simulink model "MMC_1ph_Grid_ArmLeaders_EnergyBalancing_v3_1A"  (R2024a)
settings: Solver=FixedStepDiscrete  StartTime=0.0  StopTime=1  FixedStep=Ts  RelTol=1e-3
PreLoadFcn:
  | VDC=800; N=8; C=2.2e-3; vo=100; W_nom=0.5*C*N*vo^2;
  | Larm=5e-3; Rarm=0.5; f=50;
  | Vg_rms=230; Vg_pk=Vg_rms*sqrt(2); Lg=2e-3; Rg=0.1;
  | Pstar=1500; Qstar=0;
  | fsw=1250; Ts=1e-5; Ts_ctrl=1e-4; Cf=10e-6; Rf=10;
InitFcn:
  | VDC=800; N=8; C=2.2e-3; vo=100; W_nom=0.5*C*N*vo^2;
  | Larm=5e-3; Rarm=0.5; f=50;
  | Vg_rms=230; Vg_pk=Vg_rms*sqrt(2); Lg=2e-3; Rg=0.1;
  | Pstar=1500; Qstar=0;
  | fsw=1250; Ts=1e-5; Ts_ctrl=1e-4; Cf=10e-6; Rf=10;
libraries: spsHalfBridgeMMCLib x16, spsSeriesRLCBranchLib x4, spsCurrentMeasurementLib x3, spsGroundLib x2, spsDCVoltageSourceLib x2, spsACVoltageSourceLib x1, spspowerguiLib x1, spsVoltageMeasurementLib x1
(part 1 of 2)
settings Model: Creator=Dell  LastModifiedBy=Dell
settings SolverCC: AutoInsertRateTranBlk=on

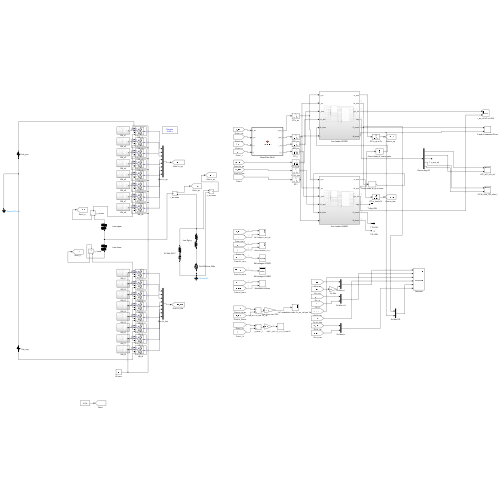
[thumbnail: Simulink's stored preview of the top-level diagram]
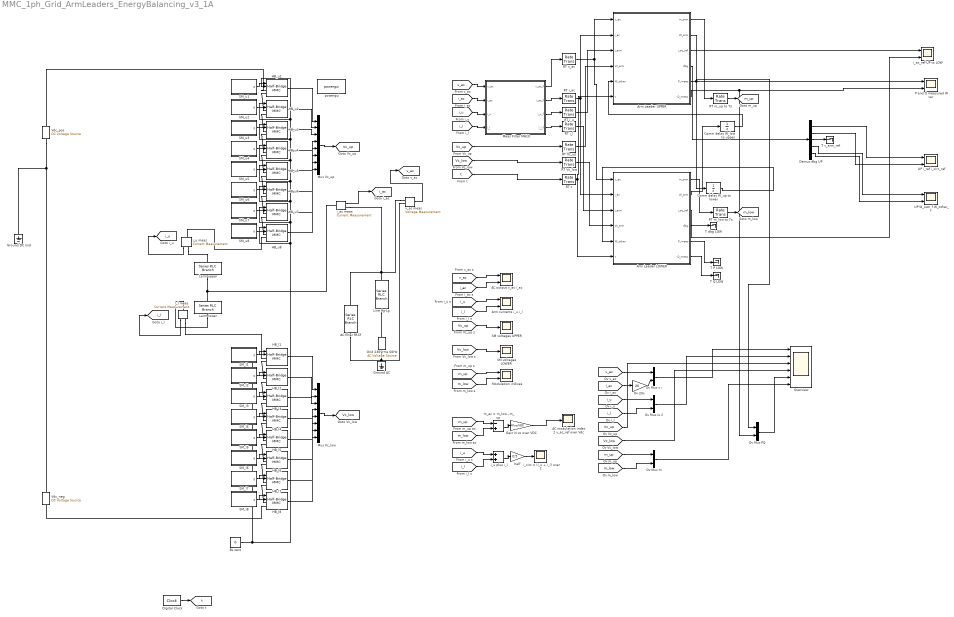
== system MMC_1ph_Grid_ArmLeaders_EnergyBalancing_v3_1A ==
  AC filter Rf-Cf : spsSeriesRLCBranchLib/Series RLC Branch  LConnTagsString=__new0  RConnTagsString=__new0  BranchType=RC  Resistance=Rf  Inductance=1e-3  SetiL0=off  InitialCurrent=0  Capacitance=Cf  Setx0=off  InitialVoltage=0  Measurements=None
  AC modulation index 2 v_ac_ref over Vdc : Scope
  AC output v_ac i_ac : Scope  NumInputPorts=2
  Arm Leader LOWER : Subsystem
  Arm Leader UPPER : Subsystem
  Arm currents i_u i_l : Scope  NumInputPorts=2
  BL zero : Constant  Value=0
  Comm delay W_low to upper : UnitDelay  InitialCondition=W_nom  SampleTime=Ts_ctrl  HasFrameUpgradeWarning=on
  Comm delay W_up to lower : UnitDelay  InitialCondition=W_nom  SampleTime=Ts_ctrl  HasFrameUpgradeWarning=on
  Demux dbg UP : Demux  Outputs=5
  Digital Clock : DigitalClock  SampleTime=Ts
  Gain N vo over VDC : Gain  Gain=N*vo/VDC
  Grid 230Vrms 50Hz : spsACVoltageSourceLib/AC Voltage Source  Amplitude=Vg_pk  Phase=0  Frequency=f  SampleTime=0  Measurements=None  BusType=swing  Pref=10e3  Qref=0  Qmin=-inf  Qmax=+inf
  Ground AC : spsGroundLib/Ground  LConnTagsString=a
  Ground DC mid : spsGroundLib/Ground  LConnTagsString=a
  HB_l{1..8} (8 alike) : spsHalfBridgeMMCLib/Half-Bridge MMC  ModelType=Switching devices  n=1  C=C  Vc_Initial=vo  Ron=1e-3  Rs=1e6  Cs=inf  Ron_Diode=1e-3  Rs_Diode=1e6  Cs_Diode=inf  Vf_Diode=1e-3  Rs_CurrentSource=inf  Ts=Ts
  HB_u{1..8} (8 alike) : spsHalfBridgeMMCLib/Half-Bridge MMC  ModelType=Switching devices  n=1  C=C  Vc_Initial=vo  Ron=1e-3  Rs=1e6  Cs=inf  Ron_Diode=1e-3  Rs_Diode=1e6  Cs_Diode=inf  Vf_Diode=1e-3  Rs_CurrentSource=inf  Ts=Ts
  Larm lower : spsSeriesRLCBranchLib/Series RLC Branch  LConnTagsString=__new0  RConnTagsString=__new0  BranchType=RL  Resistance=Rarm  Inductance=Larm  SetiL0=off  InitialCurrent=0  Capacitance=1e-6  Setx0=off  InitialVoltage=0  Measurements=None
  Larm upper : spsSeriesRLCBranchLib/Series RLC Branch  LConnTagsString=__new0  RConnTagsString=__new0  BranchType=RL  Resistance=Rarm  Inductance=Larm  SetiL0=off  InitialCurrent=0  Capacitance=1e-6  Setx0=off  InitialVoltage=0  Measurements=None
  Line Rg-Lg : spsSeriesRLCBranchLib/Series RLC Branch  LConnTagsString=__new0  RConnTagsString=__new0  BranchType=RL  Resistance=Rg  Inductance=Lg  SetiL0=off  InitialCurrent=0  Capacitance=1e-6  Setx0=off  InitialVoltage=0  Measurements=None
  Meas Filter MA10 : MATLAB Function  TreatAsAtomicUnit=on
  Modulation indices : Scope  NumInputPorts=2
  Mux Vc_low : Mux  Inputs=8
  Mux Vc_up : Mux  Inputs=8
  Ov 20x : Gain  Gain=20
  Ov Mux PQ : Mux  Inputs=2
  Ov Mux iu il : Mux  Inputs=2
  Ov Mux m : Mux  Inputs=2
  Ov Mux v i : Mux  Inputs=2
  Overview : Scope  NumInputPorts=6
  P and Q measured W var : Scope  NumInputPorts=2
  RT Vc_low : RateTransition  OutPortSampleTime=Ts_ctrl
  RT Vc_up : RateTransition  OutPortSampleTime=Ts_ctrl
  RT i_ac : RateTransition  OutPortSampleTime=Ts_ctrl
  RT i_l : RateTransition  OutPortSampleTime=Ts_ctrl
  RT i_u : RateTransition  OutPortSampleTime=Ts_ctrl
  RT m_low to Ts : RateTransition  Deterministic=off  OutPortSampleTime=Ts
  RT m_up to Ts : RateTransition  Deterministic=off  OutPortSampleTime=Ts
  RT t : RateTransition  OutPortSampleTime=Ts_ctrl
  RT v_ac : RateTransition  OutPortSampleTime=Ts_ctrl
  SM voltages LOWER : Scope
  SM voltages UPPER : Scope
  SM_l1 : Subsystem
  SM_l2 : Subsystem
  SM_l3 : Subsystem
  SM_l4 : Subsystem
  SM_l5 : Subsystem
  SM_l6 : Subsystem
  SM_l7 : Subsystem
  SM_l8 : Subsystem
  SM_u1 : Subsystem
  SM_u2 : Subsystem
  SM_u3 : Subsystem
  SM_u4 : Subsystem
  SM_u5 : Subsystem
  SM_u6 : Subsystem
  SM_u7 : Subsystem
  SM_u8 : Subsystem
  T P LOW : Terminator
  T Q LOW : Terminator
  T dbg LOW : Terminator
  T v_arm_ref : Terminator
  UP W_own_f W_other_f : Scope  NumInputPorts=2
  UP i_ref i_circ_ref : Scope  NumInputPorts=2
  Vdc_neg : spsDCVoltageSourceLib/DC Voltage Source  Amplitude=VDC/2  Measurements=None
  Vdc_pos : spsDCVoltageSourceLib/DC Voltage Source  Amplitude=VDC/2  Measurements=None
  half : Gain  Gain=0.5
  i_ac meas : spsCurrentMeasurementLib/Current Measurement  PhasorSimulation=off  OutputType=Complex  PSBequivalent=0
  i_ac_ref UP vs LOW : Scope  NumInputPorts=2
  i_circ = (i_u + i_l) over 2 : Scope
  i_l meas : spsCurrentMeasurementLib/Current Measurement  PhasorSimulation=off  OutputType=Complex  PSBequivalent=0
  i_u meas : spsCurrentMeasurementLib/Current Measurement  PhasorSimulation=off  OutputType=Complex  PSBequivalent=0
  i_u plus i_l : Sum
  m_ac = m_low - m_up : Sum  Inputs=-+
  powergui : spspowerguiLib/powergui  Priority=1  SimulationMode=Discrete  SampleTime=Ts  frequency=50  Iterations=50  frequencyindice=50  Pbase=100e6  ErrMax=1e-4  UnitsV=kV  UnitsW=MW  buscounter=0  FunctionMessages=off  echomessages=off  EnableUseOfTLC=off  CurrentSourceSwitches=off  DisableSnubberDevices=off  DisableRonSwitches=off  DisableVfSwitches=off  DisplayEquations=off  AutomaticDiscreteSolvers=off  SolverType=Tustin/Backward Euler (TBE)  Interpol=off  ExternalGateDelay=off  methode=off  Ts=100  x0status=blocks  SPID=on  SwTol=0  HookPort=off  NonlinearTolerance=1e-4  nMaxIteration=100  ContinueOnMaxIteration=off  RestoreLinks=warning  ResistiveCurrentMeasurement=off  Frange=[0:2:500]  Ylog=off  Xlog=on  ShowGrid=off  save=off  variable=ZData  structure=0  ZoomFFT=off  StartTime=0.0  cycles=1  DisplayStyle=1  fundamental=50  FreqAxis=off  MaxFrequency=1000  frequencyindicesteady=1  RmsSteady=1  display=off
  v_ac meas : spsVoltageMeasurementLib/Voltage Measurement  PhasorSimulation=off  OutputType=Complex  PSBequivalent=0
  tag scope: Vc_low=global, Vc_up=global, i_ac=global, i_l=global, i_u=global, m_low=global, m_up=global, t=global, v_ac=global
  wires:
  v_ac meas/1 -> [v_ac]
  i_ac meas/1 -> [i_ac]
  i_u meas/1 -> [i_u]
  i_l meas/1 -> [i_l]
  BL zero/1 -> HB_u1/2, HB_u2/2, HB_u3/2, HB_u4/2, HB_u5/2, HB_u6/2, HB_u7/2, HB_u8/2, HB_l1/2, HB_l2/2, HB_l3/2, HB_l4/2, HB_l5/2, HB_l6/2, HB_l7/2, HB_l8/2
  HB_u1/1 -> Mux Vc_up/1
  HB_l1/1 -> Mux Vc_low/1
  HB_u2/1 -> Mux Vc_up/2
  HB_l2/1 -> Mux Vc_low/2
  HB_u3/1 -> Mux Vc_up/3
  HB_l3/1 -> Mux Vc_low/3
  HB_u4/1 -> Mux Vc_up/4
  HB_l4/1 -> Mux Vc_low/4
  HB_u5/1 -> Mux Vc_up/5
  HB_l5/1 -> Mux Vc_low/5
  HB_u6/1 -> Mux Vc_up/6
  HB_l6/1 -> Mux Vc_low/6
  HB_u7/1 -> Mux Vc_up/7
  HB_l7/1 -> Mux Vc_low/7
  HB_u8/1 -> Mux Vc_up/8
  HB_l8/1 -> Mux Vc_low/8
  Mux Vc_up/1 -> [Vc_up]
  Mux Vc_low/1 -> [Vc_low]
  Digital Clock/1 -> [t]
  SM_u1/1(g) -> HB_u1/1
  SM_l1/1(g) -> HB_l1/1
  SM_u2/1(g) -> HB_u2/1
  SM_l2/1(g) -> HB_l2/1
  SM_u3/1(g) -> HB_u3/1
  SM_l3/1(g) -> HB_l3/1
  SM_u4/1(g) -> HB_u4/1
  SM_l4/1(g) -> HB_l4/1
  SM_u5/1(g) -> HB_u5/1
  SM_l5/1(g) -> HB_l5/1
  SM_u6/1(g) -> HB_u6/1
  SM_l6/1(g) -> HB_l6/1
  SM_u7/1(g) -> HB_u7/1
  SM_l7/1(g) -> HB_l7/1
  SM_u8/1(g) -> HB_u8/1
  SM_l8/1(g) -> HB_l8/1
  [v_ac] -> Meas Filter MA10/1(v_ac)
  [i_ac] -> Meas Filter MA10/2(i_ac)
  [i_u] -> Meas Filter MA10/3(i_u)
  [i_l] -> Meas Filter MA10/4(i_l)
  Meas Filter MA10/1(v_ac_f) -> RT v_ac/1
  Meas Filter MA10/2(i_ac_f) -> RT i_ac/1
  Meas Filter MA10/3(i_u_f) -> RT i_u/1
  Meas Filter MA10/4(i_l_f) -> RT i_l/1
  [Vc_up] -> RT Vc_up/1
  [Vc_low] -> RT Vc_low/1
  [t] -> RT t/1
  RT v_ac/1 -> Arm Leader LOWER/1(v_ac), Arm Leader UPPER/1(v_ac)
  RT i_ac/1 -> Arm Leader UPPER/2(i_ac), Arm Leader LOWER/2(i_ac)
  RT i_u/1 -> Arm Leader UPPER/3(i_arm)
  RT i_l/1 -> Arm Leader LOWER/3(i_arm)
  RT Vc_up/1 -> Arm Leader UPPER/4(Vc_arm)
  RT Vc_low/1 -> Arm Leader LOWER/4(Vc_arm)
  RT t/1 -> Arm Leader UPPER/6(t), Arm Leader LOWER/6(t)
  Arm Leader UPPER/2(W_arm) -> Comm delay W_up to lower/1
  Comm delay W_up to lower/1 -> Arm Leader LOWER/5(W_other)
  Arm Leader LOWER/2(W_arm) -> Comm delay W_low to upper/1
  Comm delay W_low to upper/1 -> Arm Leader UPPER/5(W_other)
  Arm Leader UPPER/1(m_arm) -> RT m_up to Ts/1
  RT m_up to Ts/1 -> [m_up]
  Arm Leader LOWER/1(m_arm) -> RT m_low to Ts/1
  RT m_low to Ts/1 -> [m_low]
  [v_ac] -> AC output v_ac i_ac/1
  [i_ac] -> AC output v_ac i_ac/2
  [i_u] -> Arm currents i_u i_l/1
  [i_l] -> Arm currents i_u i_l/2
  [Vc_up] -> SM voltages UPPER/1
  [Vc_low] -> SM voltages LOWER/1
  [m_up] -> Modulation indices/1
  [m_low] -> Modulation indices/2
  [m_up] -> m_ac = m_low - m_up/1
  [m_low] -> m_ac = m_low - m_up/2
  m_ac = m_low - m_up/1 -> Gain N vo over VDC/1
  Gain N vo over VDC/1 -> AC modulation index 2 v_ac_ref over Vdc/1
  [i_u] -> i_u plus i_l/1
  [i_l] -> i_u plus i_l/2
  i_u plus i_l/1 -> half/1
  half/1 -> i_circ = (i_u + i_l) over 2/1
  Arm Leader UPPER/5(P_meas) -> P and Q measured W var/1, Ov Mux PQ/1
  Arm Leader UPPER/6(Q_meas) -> P and Q measured W var/2, Ov Mux PQ/2
  Arm Leader UPPER/3(i_ac_ref) -> i_ac_ref UP vs LOW/1
  Arm Leader LOWER/3(i_ac_ref) -> i_ac_ref UP vs LOW/2
  Arm Leader UPPER/4(dbg) -> Demux dbg UP/1
  Demux dbg UP/1 -> UP i_ref i_circ_ref/1
  Demux dbg UP/2 -> UP i_ref i_circ_ref/2
  Demux dbg UP/3 -> T v_arm_ref/1
  Demux dbg UP/4 -> UP W_own_f W_other_f/1
  Demux dbg UP/5 -> UP W_own_f W_other_f/2
  Arm Leader LOWER/4(dbg) -> T dbg LOW/1
  Arm Leader LOWER/5(P_meas) -> T P LOW/1
  Arm Leader LOWER/6(Q_meas) -> T Q LOW/1
  [v_ac] -> Ov Mux v i/1
  [i_ac] -> Ov 20x/1
  Ov 20x/1 -> Ov Mux v i/2
  [i_u] -> Ov Mux iu il/1
  [i_l] -> Ov Mux iu il/2
  [m_up] -> Ov Mux m/1
  [m_low] -> Ov Mux m/2
  Ov Mux v i/1 -> Overview/1
  Ov Mux iu il/1 -> Overview/2
  [Vc_up] -> Overview/3
  [Vc_low] -> Overview/4
  Ov Mux PQ/1 -> Overview/5
  Ov Mux m/1 -> Overview/6
  connections:
  HB_u1/LConn1 -- Vdc_pos/RConn1
  Vdc_pos/LConn1 -- Ground DC mid/LConn1 -- Vdc_neg/RConn1
  HB_u1/LConn2 -- HB_u2/LConn1
  HB_l1/LConn2 -- HB_l2/LConn1
  HB_u2/LConn2 -- HB_u3/LConn1
  HB_l2/LConn2 -- HB_l3/LConn1
  HB_u3/LConn2 -- HB_u4/LConn1
  HB_l3/LConn2 -- HB_l4/LConn1
  HB_u4/LConn2 -- HB_u5/LConn1
  HB_l4/LConn2 -- HB_l5/LConn1
  HB_u5/LConn2 -- HB_u6/LConn1
  HB_l5/LConn2 -- HB_l6/LConn1
  HB_u6/LConn2 -- HB_u7/LConn1
  HB_l6/LConn2 -- HB_l7/LConn1
  HB_u7/LConn2 -- HB_u8/LConn1
  HB_l7/LConn2 -- HB_l8/LConn1
  HB_u8/LConn2 -- i_u meas/LConn1
  i_u meas/RConn1 -- Larm upper/LConn1
  Larm upper/RConn1 -- i_ac meas/LConn1 -- Larm lower/LConn1
  Larm lower/RConn1 -- i_l meas/LConn1
  i_l meas/RConn1 -- HB_l1/LConn1
  HB_l8/LConn2 -- Vdc_neg/LConn1
  v_ac meas/LConn1 -- i_ac meas/RConn1 -- Line Rg-Lg/LConn1 -- AC filter Rf-Cf/LConn1
  Line Rg-Lg/RConn1 -- Grid 230Vrms 50Hz/RConn1
  Grid 230Vrms 50Hz/LConn1 -- AC filter Rf-Cf/RConn1 -- v_ac meas/LConn2 -- Ground AC/LConn1

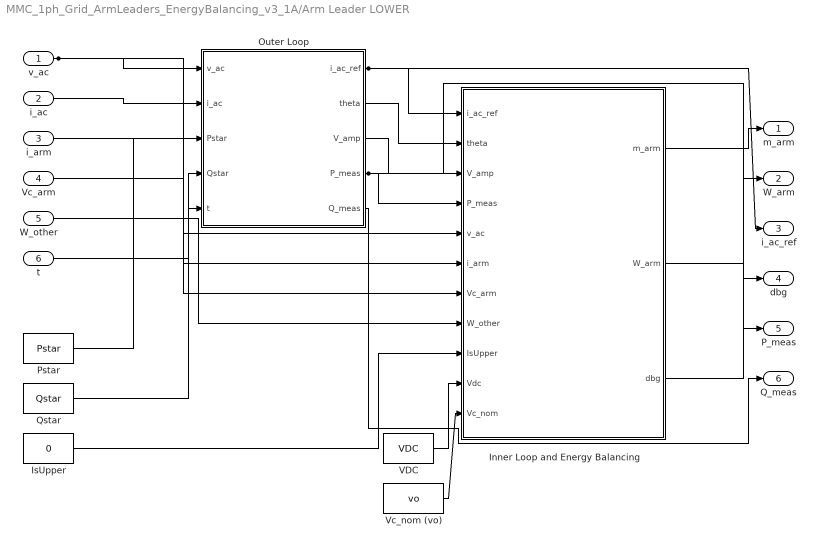
== system MMC_1ph_Grid_ArmLeaders_EnergyBalancing_v3_1A/Arm Leader LOWER ==
  v_ac : Inport
  i_ac : Inport  Port=2
  i_arm : Inport  Port=3
  Vc_arm : Inport  Port=4
  W_other : Inport  Port=5
  t : Inport  Port=6
  Inner Loop and Energy Balancing : MATLAB Function  TreatAsAtomicUnit=on
  IsUpper : Constant  Value=0
  Outer Loop : MATLAB Function  TreatAsAtomicUnit=on
  Pstar : Constant  Value=Pstar
  Qstar : Constant  Value=Qstar
  VDC : Constant  Value=VDC
  Vc_nom (vo) : Constant  Value=vo
  m_arm : Outport
  W_arm : Outport  Port=2
  i_ac_ref : Outport  Port=3
  dbg : Outport  Port=4
  P_meas : Outport  Port=5
  Q_meas : Outport  Port=6
  wires:
  v_ac/1 -> Outer Loop/1(v_ac), Inner Loop and Energy Balancing/5(v_ac)
  i_ac/1 -> Outer Loop/2(i_ac)
  Pstar/1 -> Outer Loop/3(Pstar)
  Qstar/1 -> Outer Loop/4(Qstar)
  t/1 -> Outer Loop/5(t)
  Outer Loop/1(i_ac_ref) -> Inner Loop and Energy Balancing/1(i_ac_ref), i_ac_ref/1
  Outer Loop/2(theta) -> Inner Loop and Energy Balancing/2(theta)
  Outer Loop/3(V_amp) -> Inner Loop and Energy Balancing/3(V_amp)
  Outer Loop/4(P_meas) -> Inner Loop and Energy Balancing/4(P_meas), P_meas/1
  Outer Loop/5(Q_meas) -> Q_meas/1
  i_arm/1 -> Inner Loop and Energy Balancing/6(i_arm)
  Vc_arm/1 -> Inner Loop and Energy Balancing/7(Vc_arm)
  W_other/1 -> Inner Loop and Energy Balancing/8(W_other)
  IsUpper/1 -> Inner Loop and Energy Balancing/9(IsUpper)
  VDC/1 -> Inner Loop and Energy Balancing/10(Vdc)
  Vc_nom (vo)/1 -> Inner Loop and Energy Balancing/11(Vc_nom)
  Inner Loop and Energy Balancing/1(m_arm) -> m_arm/1
  Inner Loop and Energy Balancing/2(W_arm) -> W_arm/1
  Inner Loop and Energy Balancing/3(dbg) -> dbg/1

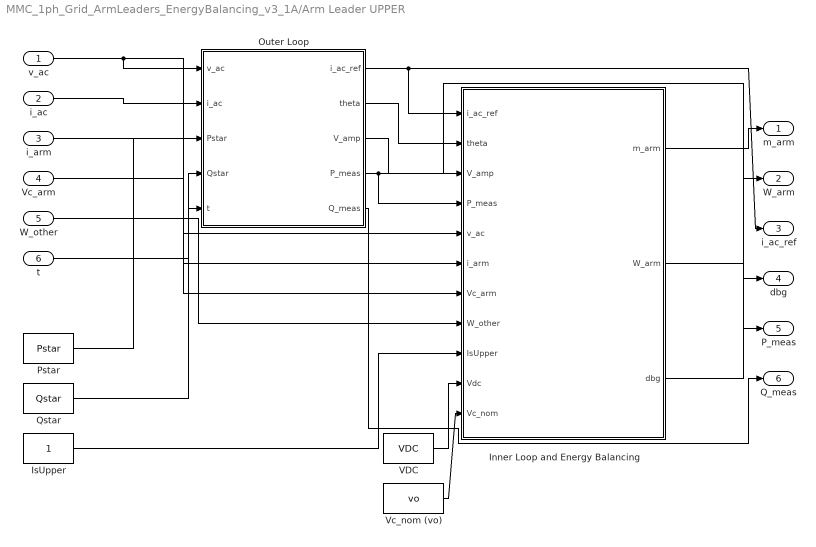
== system MMC_1ph_Grid_ArmLeaders_EnergyBalancing_v3_1A/Arm Leader UPPER ==
  v_ac : Inport
  i_ac : Inport  Port=2
  i_arm : Inport  Port=3
  Vc_arm : Inport  Port=4
  W_other : Inport  Port=5
  t : Inport  Port=6
  Inner Loop and Energy Balancing : MATLAB Function  TreatAsAtomicUnit=on
  IsUpper : Constant
  Outer Loop : MATLAB Function  TreatAsAtomicUnit=on
  Pstar : Constant  Value=Pstar
  Qstar : Constant  Value=Qstar
  VDC : Constant  Value=VDC
  Vc_nom (vo) : Constant  Value=vo
  m_arm : Outport
  W_arm : Outport  Port=2
  i_ac_ref : Outport  Port=3
  dbg : Outport  Port=4
  P_meas : Outport  Port=5
  Q_meas : Outport  Port=6
  wires:
  v_ac/1 -> Outer Loop/1(v_ac), Inner Loop and Energy Balancing/5(v_ac)
  i_ac/1 -> Outer Loop/2(i_ac)
  Pstar/1 -> Outer Loop/3(Pstar)
  Qstar/1 -> Outer Loop/4(Qstar)
  t/1 -> Outer Loop/5(t)
  Outer Loop/1(i_ac_ref) -> Inner Loop and Energy Balancing/1(i_ac_ref), i_ac_ref/1
  Outer Loop/2(theta) -> Inner Loop and Energy Balancing/2(theta)
  Outer Loop/3(V_amp) -> Inner Loop and Energy Balancing/3(V_amp)
  Outer Loop/4(P_meas) -> Inner Loop and Energy Balancing/4(P_meas), P_meas/1
  Outer Loop/5(Q_meas) -> Q_meas/1
  i_arm/1 -> Inner Loop and Energy Balancing/6(i_arm)
  Vc_arm/1 -> Inner Loop and Energy Balancing/7(Vc_arm)
  W_other/1 -> Inner Loop and Energy Balancing/8(W_other)
  IsUpper/1 -> Inner Loop and Energy Balancing/9(IsUpper)
  VDC/1 -> Inner Loop and Energy Balancing/10(Vdc)
  Vc_nom (vo)/1 -> Inner Loop and Energy Balancing/11(Vc_nom)
  Inner Loop and Energy Balancing/1(m_arm) -> m_arm/1
  Inner Loop and Energy Balancing/2(W_arm) -> W_arm/1
  Inner Loop and Energy Balancing/3(dbg) -> dbg/1

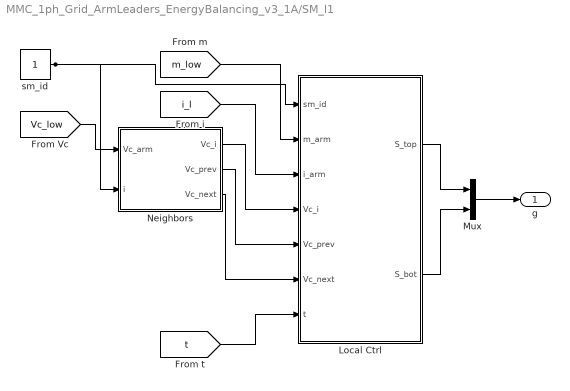
== system MMC_1ph_Grid_ArmLeaders_EnergyBalancing_v3_1A/SM_l1 ==
  Local Ctrl : MATLAB Function  TreatAsAtomicUnit=on
  Mux : Mux  Inputs=2
  Neighbors : MATLAB Function  TreatAsAtomicUnit=on
  sm_id : Constant
  g : Outport
  wires:
  [Vc_low] -> Neighbors/1(Vc_arm)
  sm_id/1 -> Neighbors/2(i), Local Ctrl/1(sm_id)
  [m_low] -> Local Ctrl/2(m_arm)
  [i_l] -> Local Ctrl/3(i_arm)
  Neighbors/1(Vc_i) -> Local Ctrl/4(Vc_i)
  Neighbors/2(Vc_prev) -> Local Ctrl/5(Vc_prev)
  Neighbors/3(Vc_next) -> Local Ctrl/6(Vc_next)
  [t] -> Local Ctrl/7(t)
  Local Ctrl/1(S_top) -> Mux/1
  Local Ctrl/2(S_bot) -> Mux/2
  Mux/1 -> g/1

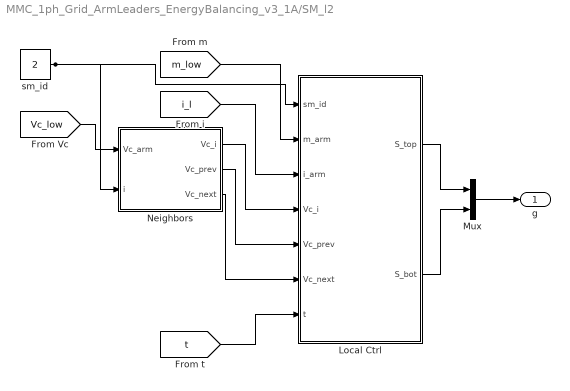
== system MMC_1ph_Grid_ArmLeaders_EnergyBalancing_v3_1A/SM_l2 ==
  Local Ctrl : MATLAB Function  TreatAsAtomicUnit=on
  Mux : Mux  Inputs=2
  Neighbors : MATLAB Function  TreatAsAtomicUnit=on
  sm_id : Constant  Value=2
  g : Outport
  wires:
  [Vc_low] -> Neighbors/1(Vc_arm)
  sm_id/1 -> Neighbors/2(i), Local Ctrl/1(sm_id)
  [m_low] -> Local Ctrl/2(m_arm)
  [i_l] -> Local Ctrl/3(i_arm)
  Neighbors/1(Vc_i) -> Local Ctrl/4(Vc_i)
  Neighbors/2(Vc_prev) -> Local Ctrl/5(Vc_prev)
  Neighbors/3(Vc_next) -> Local Ctrl/6(Vc_next)
  [t] -> Local Ctrl/7(t)
  Local Ctrl/1(S_top) -> Mux/1
  Local Ctrl/2(S_bot) -> Mux/2
  Mux/1 -> g/1

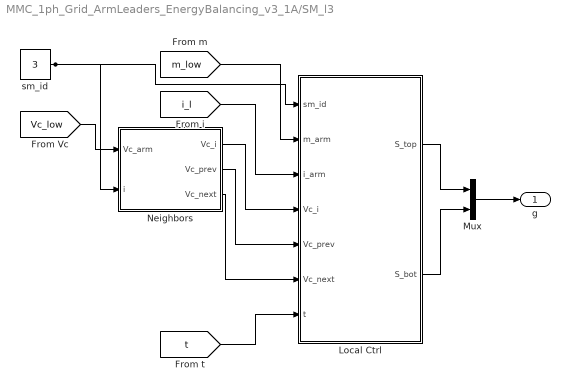
== system MMC_1ph_Grid_ArmLeaders_EnergyBalancing_v3_1A/SM_l3 ==
  Local Ctrl : MATLAB Function  TreatAsAtomicUnit=on
  Mux : Mux  Inputs=2
  Neighbors : MATLAB Function  TreatAsAtomicUnit=on
  sm_id : Constant  Value=3
  g : Outport
  wires:
  [Vc_low] -> Neighbors/1(Vc_arm)
  sm_id/1 -> Neighbors/2(i), Local Ctrl/1(sm_id)
  [m_low] -> Local Ctrl/2(m_arm)
  [i_l] -> Local Ctrl/3(i_arm)
  Neighbors/1(Vc_i) -> Local Ctrl/4(Vc_i)
  Neighbors/2(Vc_prev) -> Local Ctrl/5(Vc_prev)
  Neighbors/3(Vc_next) -> Local Ctrl/6(Vc_next)
  [t] -> Local Ctrl/7(t)
  Local Ctrl/1(S_top) -> Mux/1
  Local Ctrl/2(S_bot) -> Mux/2
  Mux/1 -> g/1

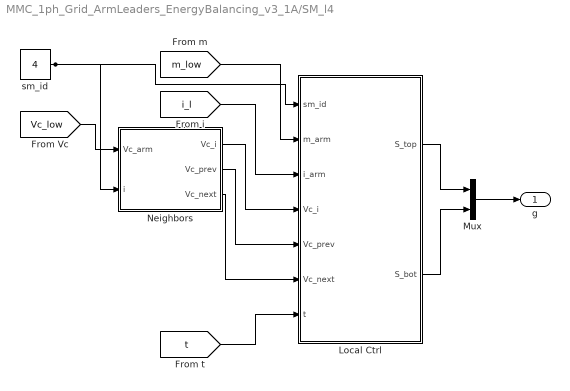
== system MMC_1ph_Grid_ArmLeaders_EnergyBalancing_v3_1A/SM_l4 ==
  Local Ctrl : MATLAB Function  TreatAsAtomicUnit=on
  Mux : Mux  Inputs=2
  Neighbors : MATLAB Function  TreatAsAtomicUnit=on
  sm_id : Constant  Value=4
  g : Outport
  wires:
  [Vc_low] -> Neighbors/1(Vc_arm)
  sm_id/1 -> Neighbors/2(i), Local Ctrl/1(sm_id)
  [m_low] -> Local Ctrl/2(m_arm)
  [i_l] -> Local Ctrl/3(i_arm)
  Neighbors/1(Vc_i) -> Local Ctrl/4(Vc_i)
  Neighbors/2(Vc_prev) -> Local Ctrl/5(Vc_prev)
  Neighbors/3(Vc_next) -> Local Ctrl/6(Vc_next)
  [t] -> Local Ctrl/7(t)
  Local Ctrl/1(S_top) -> Mux/1
  Local Ctrl/2(S_bot) -> Mux/2
  Mux/1 -> g/1

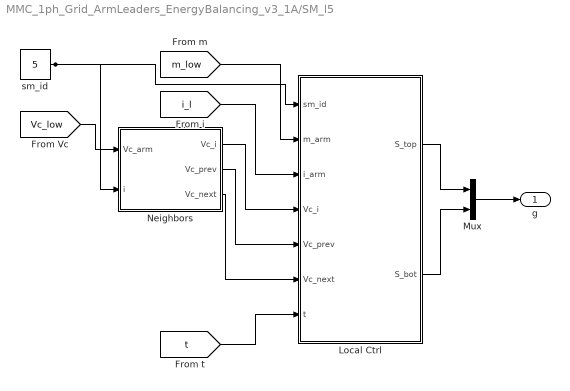
== system MMC_1ph_Grid_ArmLeaders_EnergyBalancing_v3_1A/SM_l5 ==
  Local Ctrl : MATLAB Function  TreatAsAtomicUnit=on
  Mux : Mux  Inputs=2
  Neighbors : MATLAB Function  TreatAsAtomicUnit=on
  sm_id : Constant  Value=5
  g : Outport
  wires:
  [Vc_low] -> Neighbors/1(Vc_arm)
  sm_id/1 -> Neighbors/2(i), Local Ctrl/1(sm_id)
  [m_low] -> Local Ctrl/2(m_arm)
  [i_l] -> Local Ctrl/3(i_arm)
  Neighbors/1(Vc_i) -> Local Ctrl/4(Vc_i)
  Neighbors/2(Vc_prev) -> Local Ctrl/5(Vc_prev)
  Neighbors/3(Vc_next) -> Local Ctrl/6(Vc_next)
  [t] -> Local Ctrl/7(t)
  Local Ctrl/1(S_top) -> Mux/1
  Local Ctrl/2(S_bot) -> Mux/2
  Mux/1 -> g/1

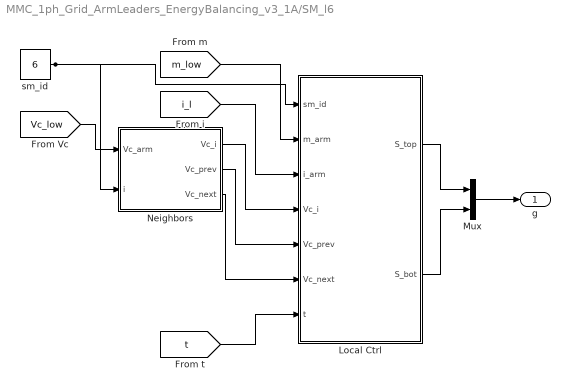
== system MMC_1ph_Grid_ArmLeaders_EnergyBalancing_v3_1A/SM_l6 ==
  Local Ctrl : MATLAB Function  TreatAsAtomicUnit=on
  Mux : Mux  Inputs=2
  Neighbors : MATLAB Function  TreatAsAtomicUnit=on
  sm_id : Constant  Value=6
  g : Outport
  wires:
  [Vc_low] -> Neighbors/1(Vc_arm)
  sm_id/1 -> Neighbors/2(i), Local Ctrl/1(sm_id)
  [m_low] -> Local Ctrl/2(m_arm)
  [i_l] -> Local Ctrl/3(i_arm)
  Neighbors/1(Vc_i) -> Local Ctrl/4(Vc_i)
  Neighbors/2(Vc_prev) -> Local Ctrl/5(Vc_prev)
  Neighbors/3(Vc_next) -> Local Ctrl/6(Vc_next)
  [t] -> Local Ctrl/7(t)
  Local Ctrl/1(S_top) -> Mux/1
  Local Ctrl/2(S_bot) -> Mux/2
  Mux/1 -> g/1

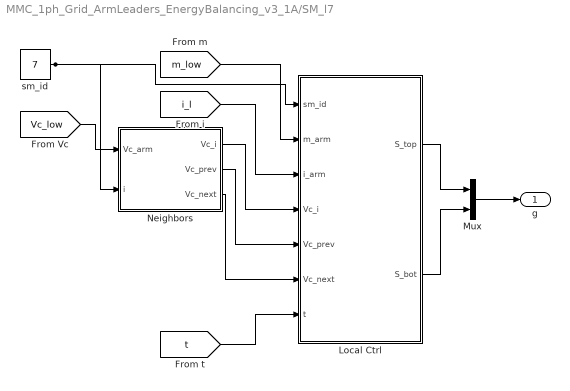
== system MMC_1ph_Grid_ArmLeaders_EnergyBalancing_v3_1A/SM_l7 ==
  Local Ctrl : MATLAB Function  TreatAsAtomicUnit=on
  Mux : Mux  Inputs=2
  Neighbors : MATLAB Function  TreatAsAtomicUnit=on
  sm_id : Constant  Value=7
  g : Outport
  wires:
  [Vc_low] -> Neighbors/1(Vc_arm)
  sm_id/1 -> Neighbors/2(i), Local Ctrl/1(sm_id)
  [m_low] -> Local Ctrl/2(m_arm)
  [i_l] -> Local Ctrl/3(i_arm)
  Neighbors/1(Vc_i) -> Local Ctrl/4(Vc_i)
  Neighbors/2(Vc_prev) -> Local Ctrl/5(Vc_prev)
  Neighbors/3(Vc_next) -> Local Ctrl/6(Vc_next)
  [t] -> Local Ctrl/7(t)
  Local Ctrl/1(S_top) -> Mux/1
  Local Ctrl/2(S_bot) -> Mux/2
  Mux/1 -> g/1

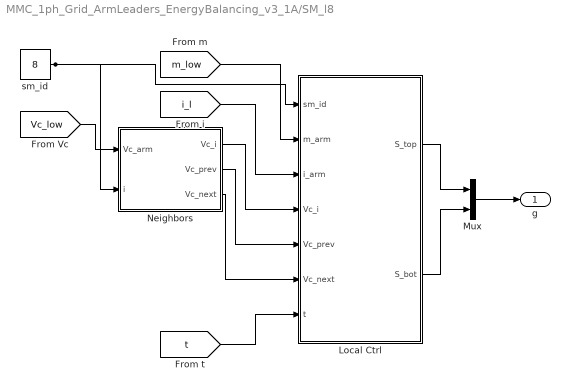
== system MMC_1ph_Grid_ArmLeaders_EnergyBalancing_v3_1A/SM_l8 ==
  Local Ctrl : MATLAB Function  TreatAsAtomicUnit=on
  Mux : Mux  Inputs=2
  Neighbors : MATLAB Function  TreatAsAtomicUnit=on
  sm_id : Constant  Value=8
  g : Outport
  wires:
  [Vc_low] -> Neighbors/1(Vc_arm)
  sm_id/1 -> Neighbors/2(i), Local Ctrl/1(sm_id)
  [m_low] -> Local Ctrl/2(m_arm)
  [i_l] -> Local Ctrl/3(i_arm)
  Neighbors/1(Vc_i) -> Local Ctrl/4(Vc_i)
  Neighbors/2(Vc_prev) -> Local Ctrl/5(Vc_prev)
  Neighbors/3(Vc_next) -> Local Ctrl/6(Vc_next)
  [t] -> Local Ctrl/7(t)
  Local Ctrl/1(S_top) -> Mux/1
  Local Ctrl/2(S_bot) -> Mux/2
  Mux/1 -> g/1

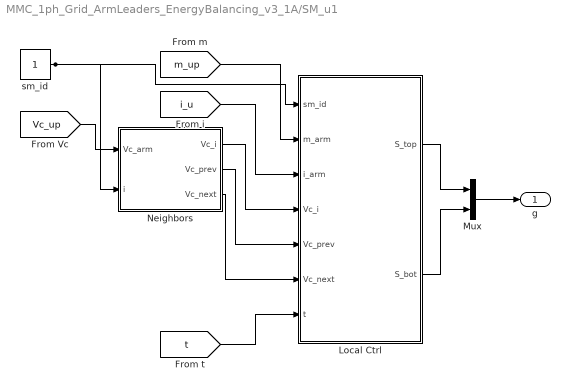
== system MMC_1ph_Grid_ArmLeaders_EnergyBalancing_v3_1A/SM_u1 ==
  Local Ctrl : MATLAB Function  TreatAsAtomicUnit=on
  Mux : Mux  Inputs=2
  Neighbors : MATLAB Function  TreatAsAtomicUnit=on
  sm_id : Constant
  g : Outport
  wires:
  [Vc_up] -> Neighbors/1(Vc_arm)
  sm_id/1 -> Neighbors/2(i), Local Ctrl/1(sm_id)
  [m_up] -> Local Ctrl/2(m_arm)
  [i_u] -> Local Ctrl/3(i_arm)
  Neighbors/1(Vc_i) -> Local Ctrl/4(Vc_i)
  Neighbors/2(Vc_prev) -> Local Ctrl/5(Vc_prev)
  Neighbors/3(Vc_next) -> Local Ctrl/6(Vc_next)
  [t] -> Local Ctrl/7(t)
  Local Ctrl/1(S_top) -> Mux/1
  Local Ctrl/2(S_bot) -> Mux/2
  Mux/1 -> g/1

== system MMC_1ph_Grid_ArmLeaders_EnergyBalancing_v3_1A/SM_u2 ==
  Local Ctrl : MATLAB Function  TreatAsAtomicUnit=on
  Mux : Mux  Inputs=2
  Neighbors : MATLAB Function  TreatAsAtomicUnit=on
  sm_id : Constant  Value=2
  g : Outport
  wires:
  [Vc_up] -> Neighbors/1(Vc_arm)
  sm_id/1 -> Neighbors/2(i), Local Ctrl/1(sm_id)
  [m_up] -> Local Ctrl/2(m_arm)
  [i_u] -> Local Ctrl/3(i_arm)
  Neighbors/1(Vc_i) -> Local Ctrl/4(Vc_i)
  Neighbors/2(Vc_prev) -> Local Ctrl/5(Vc_prev)
  Neighbors/3(Vc_next) -> Local Ctrl/6(Vc_next)
  [t] -> Local Ctrl/7(t)
  Local Ctrl/1(S_top) -> Mux/1
  Local Ctrl/2(S_bot) -> Mux/2
  Mux/1 -> g/1

== system MMC_1ph_Grid_ArmLeaders_EnergyBalancing_v3_1A/SM_u3 ==
  Local Ctrl : MATLAB Function  TreatAsAtomicUnit=on
  Mux : Mux  Inputs=2
  Neighbors : MATLAB Function  TreatAsAtomicUnit=on
  sm_id : Constant  Value=3
  g : Outport
  wires:
  [Vc_up] -> Neighbors/1(Vc_arm)
  sm_id/1 -> Neighbors/2(i), Local Ctrl/1(sm_id)
  [m_up] -> Local Ctrl/2(m_arm)
  [i_u] -> Local Ctrl/3(i_arm)
  Neighbors/1(Vc_i) -> Local Ctrl/4(Vc_i)
  Neighbors/2(Vc_prev) -> Local Ctrl/5(Vc_prev)
  Neighbors/3(Vc_next) -> Local Ctrl/6(Vc_next)
  [t] -> Local Ctrl/7(t)
  Local Ctrl/1(S_top) -> Mux/1
  Local Ctrl/2(S_bot) -> Mux/2
  Mux/1 -> g/1

== system MMC_1ph_Grid_ArmLeaders_EnergyBalancing_v3_1A/SM_u4 ==
  Local Ctrl : MATLAB Function  TreatAsAtomicUnit=on
  Mux : Mux  Inputs=2
  Neighbors : MATLAB Function  TreatAsAtomicUnit=on
  sm_id : Constant  Value=4
  g : Outport
  wires:
  [Vc_up] -> Neighbors/1(Vc_arm)
  sm_id/1 -> Neighbors/2(i), Local Ctrl/1(sm_id)
  [m_up] -> Local Ctrl/2(m_arm)
  [i_u] -> Local Ctrl/3(i_arm)
  Neighbors/1(Vc_i) -> Local Ctrl/4(Vc_i)
  Neighbors/2(Vc_prev) -> Local Ctrl/5(Vc_prev)
  Neighbors/3(Vc_next) -> Local Ctrl/6(Vc_next)
  [t] -> Local Ctrl/7(t)
  Local Ctrl/1(S_top) -> Mux/1
  Local Ctrl/2(S_bot) -> Mux/2
  Mux/1 -> g/1

== system MMC_1ph_Grid_ArmLeaders_EnergyBalancing_v3_1A/SM_u5 ==
  Local Ctrl : MATLAB Function  TreatAsAtomicUnit=on
  Mux : Mux  Inputs=2
  Neighbors : MATLAB Function  TreatAsAtomicUnit=on
  sm_id : Constant  Value=5
  g : Outport
  wires:
  [Vc_up] -> Neighbors/1(Vc_arm)
  sm_id/1 -> Neighbors/2(i), Local Ctrl/1(sm_id)
  [m_up] -> Local Ctrl/2(m_arm)
  [i_u] -> Local Ctrl/3(i_arm)
  Neighbors/1(Vc_i) -> Local Ctrl/4(Vc_i)
  Neighbors/2(Vc_prev) -> Local Ctrl/5(Vc_prev)
  Neighbors/3(Vc_next) -> Local Ctrl/6(Vc_next)
  [t] -> Local Ctrl/7(t)
  Local Ctrl/1(S_top) -> Mux/1
  Local Ctrl/2(S_bot) -> Mux/2
  Mux/1 -> g/1

== system MMC_1ph_Grid_ArmLeaders_EnergyBalancing_v3_1A/SM_u6 ==
  Local Ctrl : MATLAB Function  TreatAsAtomicUnit=on
  Mux : Mux  Inputs=2
  Neighbors : MATLAB Function  TreatAsAtomicUnit=on
  sm_id : Constant  Value=6
  g : Outport
  wires:
  [Vc_up] -> Neighbors/1(Vc_arm)
  sm_id/1 -> Neighbors/2(i), Local Ctrl/1(sm_id)
  [m_up] -> Local Ctrl/2(m_arm)
  [i_u] -> Local Ctrl/3(i_arm)
  Neighbors/1(Vc_i) -> Local Ctrl/4(Vc_i)
  Neighbors/2(Vc_prev) -> Local Ctrl/5(Vc_prev)
  Neighbors/3(Vc_next) -> Local Ctrl/6(Vc_next)
  [t] -> Local Ctrl/7(t)
  Local Ctrl/1(S_top) -> Mux/1
  Local Ctrl/2(S_bot) -> Mux/2
  Mux/1 -> g/1

== system MMC_1ph_Grid_ArmLeaders_EnergyBalancing_v3_1A/SM_u7 ==
  Local Ctrl : MATLAB Function  TreatAsAtomicUnit=on
  Mux : Mux  Inputs=2
  Neighbors : MATLAB Function  TreatAsAtomicUnit=on
  sm_id : Constant  Value=7
  g : Outport
  wires:
  [Vc_up] -> Neighbors/1(Vc_arm)
  sm_id/1 -> Neighbors/2(i), Local Ctrl/1(sm_id)
  [m_up] -> Local Ctrl/2(m_arm)
  [i_u] -> Local Ctrl/3(i_arm)
  Neighbors/1(Vc_i) -> Local Ctrl/4(Vc_i)
  Neighbors/2(Vc_prev) -> Local Ctrl/5(Vc_prev)
  Neighbors/3(Vc_next) -> Local Ctrl/6(Vc_next)
  [t] -> Local Ctrl/7(t)
  Local Ctrl/1(S_top) -> Mux/1
  Local Ctrl/2(S_bot) -> Mux/2
  Mux/1 -> g/1

== system MMC_1ph_Grid_ArmLeaders_EnergyBalancing_v3_1A/SM_u8 ==
  Local Ctrl : MATLAB Function  TreatAsAtomicUnit=on
  Mux : Mux  Inputs=2
  Neighbors : MATLAB Function  TreatAsAtomicUnit=on
  sm_id : Constant  Value=8
  g : Outport
  wires:
  [Vc_up] -> Neighbors/1(Vc_arm)
  sm_id/1 -> Neighbors/2(i), Local Ctrl/1(sm_id)
  [m_up] -> Local Ctrl/2(m_arm)
  [i_u] -> Local Ctrl/3(i_arm)
  Neighbors/1(Vc_i) -> Local Ctrl/4(Vc_i)
  Neighbors/2(Vc_prev) -> Local Ctrl/5(Vc_prev)
  Neighbors/3(Vc_next) -> Local Ctrl/6(Vc_next)
  [t] -> Local Ctrl/7(t)
  Local Ctrl/1(S_top) -> Mux/1
  Local Ctrl/2(S_bot) -> Mux/2
  Mux/1 -> g/1

== matlab function MMC_1ph_Grid_ArmLeaders_EnergyBalancing_v3_1A/SM_l2/Local Ctrl ==
  data: sm_id input; S_top output; m_arm input; i_arm input; Vc_i input; Vc_prev input; Vc_next input; t input; S_bot output
function [S_top, S_bot] = hb_sm_local_ctrl(sm_id, m_arm, i_arm, Vc_i, Vc_prev, Vc_next, t)
%#codegen
% ============ SUBMODULE LAYER : local voltage balancing + PSC-PWM ============
% Fully local: own capacitor voltage, the two ring neighbours, the arm modulation
% index, the arm current (sign only) and the time base.  No sorting and no access
% to the full Vc vector.  Executes at Ts (10 us).

N      = 8;         % SMs per arm  -> carrier phase shift (sm_id-1)/N
fsw    = 1250;      % carrier frequency per SM -> N*fsw = 10 kHz effective per arm
k_v    = 0.2;       % balancing gain (1/V)
dead   = 0.1;       % V, dead-band against chattering
Iscale = 1.0;       % A, smooth sign of the arm current

%% 1. neighbour-average consensus correction
err  = 0.5*(Vc_prev + Vc_next) - Vc_i;
if abs(err) < dead, err = 0; end
dirn = tanh(i_arm/Iscale);    % > 0 : inserting charges C  (both arms: i measured top -> bottom)
dm   = k_v*err*dirn;
m_i  = min(max(m_arm + dm, 0), 1);

%% 2. phase-shifted triangular carrier (0 -> 1 -> 0)
tau = mod(t*fsw + (sm_id - 1)/N, 1);
car = 1 - abs(2*tau - 1);

%% 3. half-bridge gating
if m_i >= car
    S_top = 1; S_bot = 0;     % insert  (+Vc)
else
    S_top = 0; S_bot = 1;     % bypass  (0 V)
end
end

== matlab function MMC_1ph_Grid_ArmLeaders_EnergyBalancing_v3_1A/SM_u3/Neighbors ==
  data: Vc_arm input; Vc_i output; i input; Vc_prev output; Vc_next output
function [Vc_i, Vc_prev, Vc_next] = get_neighbors(Vc_arm, i)
%#codegen
% Models the neighbour-to-neighbour link of the ring: returns the own capacitor
% voltage and the voltages of the previous / next (circular) neighbours.
% Only these three scalars reach the local controller.
N = length(Vc_arm);
k = min(max(round(i), 1), N);
Vc_i = Vc_arm(k);
if k == 1
    Vc_prev = Vc_arm(N);      % circular: SM1's previous neighbour is SMN
    Vc_next = Vc_arm(2);
elseif k == N
    Vc_prev = Vc_arm(N-1);
    Vc_next = Vc_arm(1);      % circular: SMN's next neighbour is SM1
else
    Vc_prev = Vc_arm(k-1);
    Vc_next = Vc_arm(k+1);
end
end

== matlab function MMC_1ph_Grid_ArmLeaders_EnergyBalancing_v3_1A/SM_u3/Local Ctrl ==
  data: sm_id input; S_top output; m_arm input; i_arm input; Vc_i input; Vc_prev input; Vc_next input; t input; S_bot output
function [S_top, S_bot] = hb_sm_local_ctrl(sm_id, m_arm, i_arm, Vc_i, Vc_prev, Vc_next, t)
%#codegen
% ============ SUBMODULE LAYER : local voltage balancing + PSC-PWM ============
% Fully local: own capacitor voltage, the two ring neighbours, the arm modulation
% index, the arm current (sign only) and the time base.  No sorting and no access
% to the full Vc vector.  Executes at Ts (10 us).

N      = 8;         % SMs per arm  -> carrier phase shift (sm_id-1)/N
fsw    = 1250;      % carrier frequency per SM -> N*fsw = 10 kHz effective per arm
k_v    = 0.2;       % balancing gain (1/V)
dead   = 0.1;       % V, dead-band against chattering
Iscale = 1.0;       % A, smooth sign of the arm current

%% 1. neighbour-average consensus correction
err  = 0.5*(Vc_prev + Vc_next) - Vc_i;
if abs(err) < dead, err = 0; end
dirn = tanh(i_arm/Iscale);    % > 0 : inserting charges C  (both arms: i measured top -> bottom)
dm   = k_v*err*dirn;
m_i  = min(max(m_arm + dm, 0), 1);

%% 2. phase-shifted triangular carrier (0 -> 1 -> 0)
tau = mod(t*fsw + (sm_id - 1)/N, 1);
car = 1 - abs(2*tau - 1);

%% 3. half-bridge gating
if m_i >= car
    S_top = 1; S_bot = 0;     % insert  (+Vc)
else
    S_top = 0; S_bot = 1;     % bypass  (0 V)
end
end

== matlab function MMC_1ph_Grid_ArmLeaders_EnergyBalancing_v3_1A/SM_l3/Neighbors ==
  data: Vc_arm input; Vc_i output; i input; Vc_prev output; Vc_next output
function [Vc_i, Vc_prev, Vc_next] = get_neighbors(Vc_arm, i)
%#codegen
% Models the neighbour-to-neighbour link of the ring: returns the own capacitor
% voltage and the voltages of the previous / next (circular) neighbours.
% Only these three scalars reach the local controller.
N = length(Vc_arm);
k = min(max(round(i), 1), N);
Vc_i = Vc_arm(k);
if k == 1
    Vc_prev = Vc_arm(N);      % circular: SM1's previous neighbour is SMN
    Vc_next = Vc_arm(2);
elseif k == N
    Vc_prev = Vc_arm(N-1);
    Vc_next = Vc_arm(1);      % circular: SMN's next neighbour is SM1
else
    Vc_prev = Vc_arm(k-1);
    Vc_next = Vc_arm(k+1);
end
end

== matlab function MMC_1ph_Grid_ArmLeaders_EnergyBalancing_v3_1A/SM_l3/Local Ctrl ==
  data: sm_id input; S_top output; m_arm input; i_arm input; Vc_i input; Vc_prev input; Vc_next input; t input; S_bot output
function [S_top, S_bot] = hb_sm_local_ctrl(sm_id, m_arm, i_arm, Vc_i, Vc_prev, Vc_next, t)
%#codegen
% ============ SUBMODULE LAYER : local voltage balancing + PSC-PWM ============
% Fully local: own capacitor voltage, the two ring neighbours, the arm modulation
% index, the arm current (sign only) and the time base.  No sorting and no access
% to the full Vc vector.  Executes at Ts (10 us).

N      = 8;         % SMs per arm  -> carrier phase shift (sm_id-1)/N
fsw    = 1250;      % carrier frequency per SM -> N*fsw = 10 kHz effective per arm
k_v    = 0.2;       % balancing gain (1/V)
dead   = 0.1;       % V, dead-band against chattering
Iscale = 1.0;       % A, smooth sign of the arm current

%% 1. neighbour-average consensus correction
err  = 0.5*(Vc_prev + Vc_next) - Vc_i;
if abs(err) < dead, err = 0; end
dirn = tanh(i_arm/Iscale);    % > 0 : inserting charges C  (both arms: i measured top -> bottom)
dm   = k_v*err*dirn;
m_i  = min(max(m_arm + dm, 0), 1);

%% 2. phase-shifted triangular carrier (0 -> 1 -> 0)
tau = mod(t*fsw + (sm_id - 1)/N, 1);
car = 1 - abs(2*tau - 1);

%% 3. half-bridge gating
if m_i >= car
    S_top = 1; S_bot = 0;     % insert  (+Vc)
else
    S_top = 0; S_bot = 1;     % bypass  (0 V)
end
end

== matlab function MMC_1ph_Grid_ArmLeaders_EnergyBalancing_v3_1A/SM_u4/Neighbors ==
  data: Vc_arm input; Vc_i output; i input; Vc_prev output; Vc_next output
function [Vc_i, Vc_prev, Vc_next] = get_neighbors(Vc_arm, i)
%#codegen
% Models the neighbour-to-neighbour link of the ring: returns the own capacitor
% voltage and the voltages of the previous / next (circular) neighbours.
% Only these three scalars reach the local controller.
N = length(Vc_arm);
k = min(max(round(i), 1), N);
Vc_i = Vc_arm(k);
if k == 1
    Vc_prev = Vc_arm(N);      % circular: SM1's previous neighbour is SMN
    Vc_next = Vc_arm(2);
elseif k == N
    Vc_prev = Vc_arm(N-1);
    Vc_next = Vc_arm(1);      % circular: SMN's next neighbour is SM1
else
    Vc_prev = Vc_arm(k-1);
    Vc_next = Vc_arm(k+1);
end
end

== matlab function MMC_1ph_Grid_ArmLeaders_EnergyBalancing_v3_1A/SM_u4/Local Ctrl ==
  data: sm_id input; S_top output; m_arm input; i_arm input; Vc_i input; Vc_prev input; Vc_next input; t input; S_bot output
function [S_top, S_bot] = hb_sm_local_ctrl(sm_id, m_arm, i_arm, Vc_i, Vc_prev, Vc_next, t)
%#codegen
% ============ SUBMODULE LAYER : local voltage balancing + PSC-PWM ============
% Fully local: own capacitor voltage, the two ring neighbours, the arm modulation
% index, the arm current (sign only) and the time base.  No sorting and no access
% to the full Vc vector.  Executes at Ts (10 us).

N      = 8;         % SMs per arm  -> carrier phase shift (sm_id-1)/N
fsw    = 1250;      % carrier frequency per SM -> N*fsw = 10 kHz effective per arm
k_v    = 0.2;       % balancing gain (1/V)
dead   = 0.1;       % V, dead-band against chattering
Iscale = 1.0;       % A, smooth sign of the arm current

%% 1. neighbour-average consensus correction
err  = 0.5*(Vc_prev + Vc_next) - Vc_i;
if abs(err) < dead, err = 0; end
dirn = tanh(i_arm/Iscale);    % > 0 : inserting charges C  (both arms: i measured top -> bottom)
dm   = k_v*err*dirn;
m_i  = min(max(m_arm + dm, 0), 1);

%% 2. phase-shifted triangular carrier (0 -> 1 -> 0)
tau = mod(t*fsw + (sm_id - 1)/N, 1);
car = 1 - abs(2*tau - 1);

%% 3. half-bridge gating
if m_i >= car
    S_top = 1; S_bot = 0;     % insert  (+Vc)
else
    S_top = 0; S_bot = 1;     % bypass  (0 V)
end
end

== matlab function MMC_1ph_Grid_ArmLeaders_EnergyBalancing_v3_1A/SM_l4/Neighbors ==
  data: Vc_arm input; Vc_i output; i input; Vc_prev output; Vc_next output
function [Vc_i, Vc_prev, Vc_next] = get_neighbors(Vc_arm, i)
%#codegen
% Models the neighbour-to-neighbour link of the ring: returns the own capacitor
% voltage and the voltages of the previous / next (circular) neighbours.
% Only these three scalars reach the local controller.
N = length(Vc_arm);
k = min(max(round(i), 1), N);
Vc_i = Vc_arm(k);
if k == 1
    Vc_prev = Vc_arm(N);      % circular: SM1's previous neighbour is SMN
    Vc_next = Vc_arm(2);
elseif k == N
    Vc_prev = Vc_arm(N-1);
    Vc_next = Vc_arm(1);      % circular: SMN's next neighbour is SM1
else
    Vc_prev = Vc_arm(k-1);
    Vc_next = Vc_arm(k+1);
end
end

== matlab function MMC_1ph_Grid_ArmLeaders_EnergyBalancing_v3_1A/SM_u1/Local Ctrl ==
  data: sm_id input; S_top output; m_arm input; i_arm input; Vc_i input; Vc_prev input; Vc_next input; t input; S_bot output
function [S_top, S_bot] = hb_sm_local_ctrl(sm_id, m_arm, i_arm, Vc_i, Vc_prev, Vc_next, t)
%#codegen
% ============ SUBMODULE LAYER : local voltage balancing + PSC-PWM ============
% Fully local: own capacitor voltage, the two ring neighbours, the arm modulation
% index, the arm current (sign only) and the time base.  No sorting and no access
% to the full Vc vector.  Executes at Ts (10 us).

N      = 8;         % SMs per arm  -> carrier phase shift (sm_id-1)/N
fsw    = 1250;      % carrier frequency per SM -> N*fsw = 10 kHz effective per arm
k_v    = 0.2;       % balancing gain (1/V)
dead   = 0.1;       % V, dead-band against chattering
Iscale = 1.0;       % A, smooth sign of the arm current

%% 1. neighbour-average consensus correction
err  = 0.5*(Vc_prev + Vc_next) - Vc_i;
if abs(err) < dead, err = 0; end
dirn = tanh(i_arm/Iscale);    % > 0 : inserting charges C  (both arms: i measured top -> bottom)
dm   = k_v*err*dirn;
m_i  = min(max(m_arm + dm, 0), 1);

%% 2. phase-shifted triangular carrier (0 -> 1 -> 0)
tau = mod(t*fsw + (sm_id - 1)/N, 1);
car = 1 - abs(2*tau - 1);

%% 3. half-bridge gating
if m_i >= car
    S_top = 1; S_bot = 0;     % insert  (+Vc)
else
    S_top = 0; S_bot = 1;     % bypass  (0 V)
end
end

== matlab function MMC_1ph_Grid_ArmLeaders_EnergyBalancing_v3_1A/SM_l4/Local Ctrl ==
  data: sm_id input; S_top output; m_arm input; i_arm input; Vc_i input; Vc_prev input; Vc_next input; t input; S_bot output
function [S_top, S_bot] = hb_sm_local_ctrl(sm_id, m_arm, i_arm, Vc_i, Vc_prev, Vc_next, t)
%#codegen
% ============ SUBMODULE LAYER : local voltage balancing + PSC-PWM ============
% Fully local: own capacitor voltage, the two ring neighbours, the arm modulation
% index, the arm current (sign only) and the time base.  No sorting and no access
% to the full Vc vector.  Executes at Ts (10 us).

N      = 8;         % SMs per arm  -> carrier phase shift (sm_id-1)/N
fsw    = 1250;      % carrier frequency per SM -> N*fsw = 10 kHz effective per arm
k_v    = 0.2;       % balancing gain (1/V)
dead   = 0.1;       % V, dead-band against chattering
Iscale = 1.0;       % A, smooth sign of the arm current

%% 1. neighbour-average consensus correction
err  = 0.5*(Vc_prev + Vc_next) - Vc_i;
if abs(err) < dead, err = 0; end
dirn = tanh(i_arm/Iscale);    % > 0 : inserting charges C  (both arms: i measured top -> bottom)
dm   = k_v*err*dirn;
m_i  = min(max(m_arm + dm, 0), 1);

%% 2. phase-shifted triangular carrier (0 -> 1 -> 0)
tau = mod(t*fsw + (sm_id - 1)/N, 1);
car = 1 - abs(2*tau - 1);

%% 3. half-bridge gating
if m_i >= car
    S_top = 1; S_bot = 0;     % insert  (+Vc)
else
    S_top = 0; S_bot = 1;     % bypass  (0 V)
end
end

== matlab function MMC_1ph_Grid_ArmLeaders_EnergyBalancing_v3_1A/SM_u5/Neighbors ==
  data: Vc_arm input; Vc_i output; i input; Vc_prev output; Vc_next output
function [Vc_i, Vc_prev, Vc_next] = get_neighbors(Vc_arm, i)
%#codegen
% Models the neighbour-to-neighbour link of the ring: returns the own capacitor
% voltage and the voltages of the previous / next (circular) neighbours.
% Only these three scalars reach the local controller.
N = length(Vc_arm);
k = min(max(round(i), 1), N);
Vc_i = Vc_arm(k);
if k == 1
    Vc_prev = Vc_arm(N);      % circular: SM1's previous neighbour is SMN
    Vc_next = Vc_arm(2);
elseif k == N
    Vc_prev = Vc_arm(N-1);
    Vc_next = Vc_arm(1);      % circular: SMN's next neighbour is SM1
else
    Vc_prev = Vc_arm(k-1);
    Vc_next = Vc_arm(k+1);
end
end

== matlab function MMC_1ph_Grid_ArmLeaders_EnergyBalancing_v3_1A/SM_u5/Local Ctrl ==
  data: sm_id input; S_top output; m_arm input; i_arm input; Vc_i input; Vc_prev input; Vc_next input; t input; S_bot output
function [S_top, S_bot] = hb_sm_local_ctrl(sm_id, m_arm, i_arm, Vc_i, Vc_prev, Vc_next, t)
%#codegen
% ============ SUBMODULE LAYER : local voltage balancing + PSC-PWM ============
% Fully local: own capacitor voltage, the two ring neighbours, the arm modulation
% index, the arm current (sign only) and the time base.  No sorting and no access
% to the full Vc vector.  Executes at Ts (10 us).

N      = 8;         % SMs per arm  -> carrier phase shift (sm_id-1)/N
fsw    = 1250;      % carrier frequency per SM -> N*fsw = 10 kHz effective per arm
k_v    = 0.2;       % balancing gain (1/V)
dead   = 0.1;       % V, dead-band against chattering
Iscale = 1.0;       % A, smooth sign of the arm current

%% 1. neighbour-average consensus correction
err  = 0.5*(Vc_prev + Vc_next) - Vc_i;
if abs(err) < dead, err = 0; end
dirn = tanh(i_arm/Iscale);    % > 0 : inserting charges C  (both arms: i measured top -> bottom)
dm   = k_v*err*dirn;
m_i  = min(max(m_arm + dm, 0), 1);

%% 2. phase-shifted triangular carrier (0 -> 1 -> 0)
tau = mod(t*fsw + (sm_id - 1)/N, 1);
car = 1 - abs(2*tau - 1);

%% 3. half-bridge gating
if m_i >= car
    S_top = 1; S_bot = 0;     % insert  (+Vc)
else
    S_top = 0; S_bot = 1;     % bypass  (0 V)
end
end

== matlab function MMC_1ph_Grid_ArmLeaders_EnergyBalancing_v3_1A/SM_l5/Neighbors ==
  data: Vc_arm input; Vc_i output; i input; Vc_prev output; Vc_next output
function [Vc_i, Vc_prev, Vc_next] = get_neighbors(Vc_arm, i)
%#codegen
% Models the neighbour-to-neighbour link of the ring: returns the own capacitor
% voltage and the voltages of the previous / next (circular) neighbours.
% Only these three scalars reach the local controller.
N = length(Vc_arm);
k = min(max(round(i), 1), N);
Vc_i = Vc_arm(k);
if k == 1
    Vc_prev = Vc_arm(N);      % circular: SM1's previous neighbour is SMN
    Vc_next = Vc_arm(2);
elseif k == N
    Vc_prev = Vc_arm(N-1);
    Vc_next = Vc_arm(1);      % circular: SMN's next neighbour is SM1
else
    Vc_prev = Vc_arm(k-1);
    Vc_next = Vc_arm(k+1);
end
end

== matlab function MMC_1ph_Grid_ArmLeaders_EnergyBalancing_v3_1A/SM_l5/Local Ctrl ==
  data: sm_id input; S_top output; m_arm input; i_arm input; Vc_i input; Vc_prev input; Vc_next input; t input; S_bot output
function [S_top, S_bot] = hb_sm_local_ctrl(sm_id, m_arm, i_arm, Vc_i, Vc_prev, Vc_next, t)
%#codegen
% ============ SUBMODULE LAYER : local voltage balancing + PSC-PWM ============
% Fully local: own capacitor voltage, the two ring neighbours, the arm modulation
% index, the arm current (sign only) and the time base.  No sorting and no access
% to the full Vc vector.  Executes at Ts (10 us).

N      = 8;         % SMs per arm  -> carrier phase shift (sm_id-1)/N
fsw    = 1250;      % carrier frequency per SM -> N*fsw = 10 kHz effective per arm
k_v    = 0.2;       % balancing gain (1/V)
dead   = 0.1;       % V, dead-band against chattering
Iscale = 1.0;       % A, smooth sign of the arm current

%% 1. neighbour-average consensus correction
err  = 0.5*(Vc_prev + Vc_next) - Vc_i;
if abs(err) < dead, err = 0; end
dirn = tanh(i_arm/Iscale);    % > 0 : inserting charges C  (both arms: i measured top -> bottom)
dm   = k_v*err*dirn;
m_i  = min(max(m_arm + dm, 0), 1);

%% 2. phase-shifted triangular carrier (0 -> 1 -> 0)
tau = mod(t*fsw + (sm_id - 1)/N, 1);
car = 1 - abs(2*tau - 1);

%% 3. half-bridge gating
if m_i >= car
    S_top = 1; S_bot = 0;     % insert  (+Vc)
else
    S_top = 0; S_bot = 1;     % bypass  (0 V)
end
end

== matlab function MMC_1ph_Grid_ArmLeaders_EnergyBalancing_v3_1A/SM_u6/Neighbors ==
  data: Vc_arm input; Vc_i output; i input; Vc_prev output; Vc_next output
function [Vc_i, Vc_prev, Vc_next] = get_neighbors(Vc_arm, i)
%#codegen
% Models the neighbour-to-neighbour link of the ring: returns the own capacitor
% voltage and the voltages of the previous / next (circular) neighbours.
% Only these three scalars reach the local controller.
N = length(Vc_arm);
k = min(max(round(i), 1), N);
Vc_i = Vc_arm(k);
if k == 1
    Vc_prev = Vc_arm(N);      % circular: SM1's previous neighbour is SMN
    Vc_next = Vc_arm(2);
elseif k == N
    Vc_prev = Vc_arm(N-1);
    Vc_next = Vc_arm(1);      % circular: SMN's next neighbour is SM1
else
    Vc_prev = Vc_arm(k-1);
    Vc_next = Vc_arm(k+1);
end
end

== matlab function MMC_1ph_Grid_ArmLeaders_EnergyBalancing_v3_1A/SM_u6/Local Ctrl ==
  data: sm_id input; S_top output; m_arm input; i_arm input; Vc_i input; Vc_prev input; Vc_next input; t input; S_bot output
function [S_top, S_bot] = hb_sm_local_ctrl(sm_id, m_arm, i_arm, Vc_i, Vc_prev, Vc_next, t)
%#codegen
% ============ SUBMODULE LAYER : local voltage balancing + PSC-PWM ============
% Fully local: own capacitor voltage, the two ring neighbours, the arm modulation
% index, the arm current (sign only) and the time base.  No sorting and no access
% to the full Vc vector.  Executes at Ts (10 us).

N      = 8;         % SMs per arm  -> carrier phase shift (sm_id-1)/N
fsw    = 1250;      % carrier frequency per SM -> N*fsw = 10 kHz effective per arm
k_v    = 0.2;       % balancing gain (1/V)
dead   = 0.1;       % V, dead-band against chattering
Iscale = 1.0;       % A, smooth sign of the arm current

%% 1. neighbour-average consensus correction
err  = 0.5*(Vc_prev + Vc_next) - Vc_i;
if abs(err) < dead, err = 0; end
dirn = tanh(i_arm/Iscale);    % > 0 : inserting charges C  (both arms: i measured top -> bottom)
dm   = k_v*err*dirn;
m_i  = min(max(m_arm + dm, 0), 1);

%% 2. phase-shifted triangular carrier (0 -> 1 -> 0)
tau = mod(t*fsw + (sm_id - 1)/N, 1);
car = 1 - abs(2*tau - 1);

%% 3. half-bridge gating
if m_i >= car
    S_top = 1; S_bot = 0;     % insert  (+Vc)
else
    S_top = 0; S_bot = 1;     % bypass  (0 V)
end
end

== matlab function MMC_1ph_Grid_ArmLeaders_EnergyBalancing_v3_1A/SM_l6/Neighbors ==
  data: Vc_arm input; Vc_i output; i input; Vc_prev output; Vc_next output
function [Vc_i, Vc_prev, Vc_next] = get_neighbors(Vc_arm, i)
%#codegen
% Models the neighbour-to-neighbour link of the ring: returns the own capacitor
% voltage and the voltages of the previous / next (circular) neighbours.
% Only these three scalars reach the local controller.
N = length(Vc_arm);
k = min(max(round(i), 1), N);
Vc_i = Vc_arm(k);
if k == 1
    Vc_prev = Vc_arm(N);      % circular: SM1's previous neighbour is SMN
    Vc_next = Vc_arm(2);
elseif k == N
    Vc_prev = Vc_arm(N-1);
    Vc_next = Vc_arm(1);      % circular: SMN's next neighbour is SM1
else
    Vc_prev = Vc_arm(k-1);
    Vc_next = Vc_arm(k+1);
end
end

== matlab function MMC_1ph_Grid_ArmLeaders_EnergyBalancing_v3_1A/SM_l6/Local Ctrl ==
  data: sm_id input; S_top output; m_arm input; i_arm input; Vc_i input; Vc_prev input; Vc_next input; t input; S_bot output
function [S_top, S_bot] = hb_sm_local_ctrl(sm_id, m_arm, i_arm, Vc_i, Vc_prev, Vc_next, t)
%#codegen
% ============ SUBMODULE LAYER : local voltage balancing + PSC-PWM ============
% Fully local: own capacitor voltage, the two ring neighbours, the arm modulation
% index, the arm current (sign only) and the time base.  No sorting and no access
% to the full Vc vector.  Executes at Ts (10 us).

N      = 8;         % SMs per arm  -> carrier phase shift (sm_id-1)/N
fsw    = 1250;      % carrier frequency per SM -> N*fsw = 10 kHz effective per arm
k_v    = 0.2;       % balancing gain (1/V)
dead   = 0.1;       % V, dead-band against chattering
Iscale = 1.0;       % A, smooth sign of the arm current

%% 1. neighbour-average consensus correction
err  = 0.5*(Vc_prev + Vc_next) - Vc_i;
if abs(err) < dead, err = 0; end
dirn = tanh(i_arm/Iscale);    % > 0 : inserting charges C  (both arms: i measured top -> bottom)
dm   = k_v*err*dirn;
m_i  = min(max(m_arm + dm, 0), 1);

%% 2. phase-shifted triangular carrier (0 -> 1 -> 0)
tau = mod(t*fsw + (sm_id - 1)/N, 1);
car = 1 - abs(2*tau - 1);

%% 3. half-bridge gating
if m_i >= car
    S_top = 1; S_bot = 0;     % insert  (+Vc)
else
    S_top = 0; S_bot = 1;     % bypass  (0 V)
end
end

== matlab function MMC_1ph_Grid_ArmLeaders_EnergyBalancing_v3_1A/SM_u7/Neighbors ==
  data: Vc_arm input; Vc_i output; i input; Vc_prev output; Vc_next output
function [Vc_i, Vc_prev, Vc_next] = get_neighbors(Vc_arm, i)
%#codegen
% Models the neighbour-to-neighbour link of the ring: returns the own capacitor
% voltage and the voltages of the previous / next (circular) neighbours.
% Only these three scalars reach the local controller.
N = length(Vc_arm);
k = min(max(round(i), 1), N);
Vc_i = Vc_arm(k);
if k == 1
    Vc_prev = Vc_arm(N);      % circular: SM1's previous neighbour is SMN
    Vc_next = Vc_arm(2);
elseif k == N
    Vc_prev = Vc_arm(N-1);
    Vc_next = Vc_arm(1);      % circular: SMN's next neighbour is SM1
else
    Vc_prev = Vc_arm(k-1);
    Vc_next = Vc_arm(k+1);
end
end

== matlab function MMC_1ph_Grid_ArmLeaders_EnergyBalancing_v3_1A/SM_u7/Local Ctrl ==
  data: sm_id input; S_top output; m_arm input; i_arm input; Vc_i input; Vc_prev input; Vc_next input; t input; S_bot output
function [S_top, S_bot] = hb_sm_local_ctrl(sm_id, m_arm, i_arm, Vc_i, Vc_prev, Vc_next, t)
%#codegen
% ============ SUBMODULE LAYER : local voltage balancing + PSC-PWM ============
% Fully local: own capacitor voltage, the two ring neighbours, the arm modulation
% index, the arm current (sign only) and the time base.  No sorting and no access
% to the full Vc vector.  Executes at Ts (10 us).

N      = 8;         % SMs per arm  -> carrier phase shift (sm_id-1)/N
fsw    = 1250;      % carrier frequency per SM -> N*fsw = 10 kHz effective per arm
k_v    = 0.2;       % balancing gain (1/V)
dead   = 0.1;       % V, dead-band against chattering
Iscale = 1.0;       % A, smooth sign of the arm current

%% 1. neighbour-average consensus correction
err  = 0.5*(Vc_prev + Vc_next) - Vc_i;
if abs(err) < dead, err = 0; end
dirn = tanh(i_arm/Iscale);    % > 0 : inserting charges C  (both arms: i measured top -> bottom)
dm   = k_v*err*dirn;
m_i  = min(max(m_arm + dm, 0), 1);

%% 2. phase-shifted triangular carrier (0 -> 1 -> 0)
tau = mod(t*fsw + (sm_id - 1)/N, 1);
car = 1 - abs(2*tau - 1);

%% 3. half-bridge gating
if m_i >= car
    S_top = 1; S_bot = 0;     % insert  (+Vc)
else
    S_top = 0; S_bot = 1;     % bypass  (0 V)
end
end

== matlab function MMC_1ph_Grid_ArmLeaders_EnergyBalancing_v3_1A/SM_u1/Neighbors ==
  data: Vc_arm input; Vc_i output; i input; Vc_prev output; Vc_next output
function [Vc_i, Vc_prev, Vc_next] = get_neighbors(Vc_arm, i)
%#codegen
% Models the neighbour-to-neighbour link of the ring: returns the own capacitor
% voltage and the voltages of the previous / next (circular) neighbours.
% Only these three scalars reach the local controller.
N = length(Vc_arm);
k = min(max(round(i), 1), N);
Vc_i = Vc_arm(k);
if k == 1
    Vc_prev = Vc_arm(N);      % circular: SM1's previous neighbour is SMN
    Vc_next = Vc_arm(2);
elseif k == N
    Vc_prev = Vc_arm(N-1);
    Vc_next = Vc_arm(1);      % circular: SMN's next neighbour is SM1
else
    Vc_prev = Vc_arm(k-1);
    Vc_next = Vc_arm(k+1);
end
end

== matlab function MMC_1ph_Grid_ArmLeaders_EnergyBalancing_v3_1A/SM_l7/Neighbors ==
  data: Vc_arm input; Vc_i output; i input; Vc_prev output; Vc_next output
function [Vc_i, Vc_prev, Vc_next] = get_neighbors(Vc_arm, i)
%#codegen
% Models the neighbour-to-neighbour link of the ring: returns the own capacitor
% voltage and the voltages of the previous / next (circular) neighbours.
% Only these three scalars reach the local controller.
N = length(Vc_arm);
k = min(max(round(i), 1), N);
Vc_i = Vc_arm(k);
if k == 1
    Vc_prev = Vc_arm(N);      % circular: SM1's previous neighbour is SMN
    Vc_next = Vc_arm(2);
elseif k == N
    Vc_prev = Vc_arm(N-1);
    Vc_next = Vc_arm(1);      % circular: SMN's next neighbour is SM1
else
    Vc_prev = Vc_arm(k-1);
    Vc_next = Vc_arm(k+1);
end
end
